simulink model "pwm_test"  (Simulink 7.4)
settings: Solver=FixedStepDiscrete  StartTime=0.0  StopTime=10  FixedStep=0.001  MaxStep=Ts  RelTol=1e-3
libraries: dsPICdrivers x4
settings Model: Creator=Administrator  LastModifiedBy=ELMAY  BufferReuse=off
settings DataIOCC: LimitDataPoints=off  SignalLoggingName=sigsout
settings OptimizationCC: BlockReduction=off  BooleanDataType=off  InlineInvariantSignals=on  OptimizeBlockIOStorage=off  BufferReuse=off  ExpressionFolding=off  LocalBlockOutputs=off  InitFltsAndDblsToZero=on  OptimizeModelRefInitCode=on  LifeSpan=1
settings DebuggingCC: SaveWithParameterizedLinksMsg=none  CheckExecutionContextPreStartOutputMsg=on  CheckExecutionContextRuntimeOutputMsg=on
settings HardwareCC: ProdBitPerInt=16  ProdEndianess=LittleEndian  ProdWordSize=16  ProdHWDeviceType=16-bit Generic  TargetHWDeviceType=32-bit Generic
settings RTWCC: SystemTargetFile=dspic.tlc  MakeCommand=make_CreateMPLAB  TemplateMakefile=dspic_pic30_gcc.tmf  PostCodeGenCommand=dsPIC_Compile()  Description=Embedded Target for Microchip dsPIC (real-time)  ProcessScript=dspic_make_rtw_hook
settings CodeAppCC: IgnoreCustomStorageClasses=off
settings STFCustomTargetCC: TargetFcnLib=ansi_tfl_tmw.mat  IncludeMdlTerminateFcn=off  CombineOutputUpdateFcns=on  ERTCustomFileBanners=on  SupportNonInlinedSFcns=off  CPPClassGenCompliant=on  SystemTargetFile=dspic.tlc
settings ERTTargetCC: TargetFcnLib=ansi_tfl_tmw.mat  MultiwordLength=2048  ParMdlRefBuildCompliant=off  CompOptLevelCompliant=off  IncludeMdlTerminateFcn=off  ERTFirstTimeCompliant=off  SupportContinuousTime=on  ModelStepFunctionPrototypeControlCompliant=off  ExtMode=on  ExtModeMexFile=ext_serial_win32_comm  InlinedParameterPlacement=NonHierarchical  ERTSrcFileBannerTemplate=dsPIC_code_template.cgt  ERTHdrFileBannerTemplate=dsPIC_code_template.cgt  ERTDataSrcFileTemplate=dsPIC_code_template.cgt  ERTDataHdrFileTemplate=dsPIC_code_template.cgt  ERTCustomFileTemplate=dsPIC_main.tlc  ConvertIfToSwitch=off
settings CustomProperty: DataType=string  Value=D:\PROGRA~1\MATLAB\R2009b\bin\win32\gmake

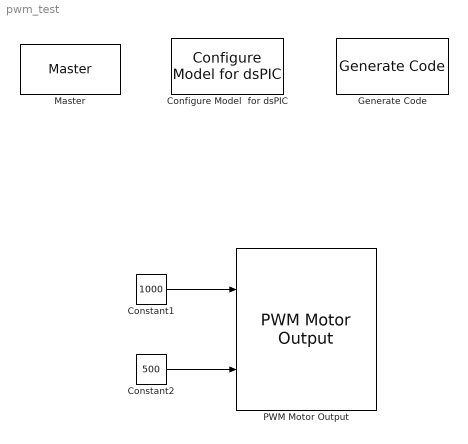
== system pwm_test ==
  Configure Model  for dsPIC : dsPICdrivers/Simulink Configuration/Configure Model  for dsPIC
  Constant1 : Constant  Value=1000  OutDataTypeMode=uint16  OutDataType=sfix(16)  OutScaling=2^0  OutDataTypeStr=uint16  SampleTime=.01
  Constant2 : Constant  Value=500  OutDataTypeMode=uint16  OutDataType=sfix(16)  OutScaling=2^0  OutDataTypeStr=uint16  SampleTime=.01
  Generate Code : dsPICdrivers/Simulink Configuration/Generate Code
  Master : dsPICdrivers/Master  Tag=dsPIC_MASTER  Priority=1  TimeStepType=Timer1  picType=30f3010  fcy=2.5e6  Quartz_33f=5e6  PLLActive_33f=off  fcyDesired_33f=0  tmr1="[1  2499  0]"  tmr1Info="Time Step : 0.001  ;   Error : 0%  PR1=2499"  tmr2345="[0  0  0  0]"  tmr2345cfg=[-1 -1 -1 -1]  IOautoConf=on  typePort="[ 0  0  0  0  0  0  0  0  0  0  0  0  0  0  0  0  0  0  0  0  0  0  0  0  0  0  0  0  0  0  0  0  0  0  0  0  0  0  0  0  0  0  0  0  0  0  0  0  0  0  0  0  0  0  0  0  0  0  0  0  0  0  0  0  0  0  0  0  0  0  0  0  0  0  0  0  0  0  0  0  0  0  0  0  0  0  0  0  0  0  0  0  0  0  0  0  0  0  0  0  0  0  0  0  0  0  0  0  0  0  0  0 ]"  TRIS="[ 65535  65535  65535  65535  65535  65535  65535 ]"  ADPCFG=0  MasterBusyPort=None  MasterOverloadPort=None  FOSC=HS  ClockSwitchMonitor=Both disabled  TempProtection_33f=TEMP_ON  FPBOR=PBOR_OFF  PWRT=PWRT_OFF  MCLR=MCLR_EN  ICD=ICS_PGD1  JTAGEN=JTAGEN_OFF  PowerSave=off  OverrideFcy=off  NewFcy=1e6  PR2345="[65535  65535  65535  65535]"
  PWM Motor Output : dsPICdrivers/Peripheral I//O/PWM Motor Output  Tag=dsPIC_PWM_Motor  Priority=5  PWMref=1  PWM12=1  InputEnableChk=off  InputPeriodeChk=on  Channel=[1]  TPeriode=0.001  PrescalerValue=1  PeriodeInteger=1250  MaxName='PWM'  Centered=on  HChannelON=off  Info="Nbr Bits : 11.2877  ||  PWM = 2500  ||  Prescaler = 1"  Delay=0  IntPriority=5  nbrPwmChannelPIC=3  Status=OK  DeadTimePrescaleA=0  DeadTimePrescaleB=0  DeadTimeInfo=Dead Time A = 0  DTPWM1a=Prescaler A  DTPWM1i=Prescaler A  DTPWM2a=Prescaler A  DTPWM2i=Prescaler A  DTPWM3a=Prescaler A  DTPWM3i=Prescaler A  DTPWM4a=Prescaler A  DTPWM4i=Prescaler A  DTCON1=0  DTCON2=0
  wires:
  Constant1/1 -> PWM Motor Output/1
  Constant2/1 -> PWM Motor Output/2
